simulink model "strapnav"  (Simulink 7.9)
settings: Solver=ode45  StartTime=0.0  StopTime=10.0  RelTol=1e-3
undefined symbols (not defined in the file or in its folder): dcm2lat, dcm2lon
libraries: simulink x2, strapnavlib x1
settings Model: Creator=mcar  LastModifiedBy=1104070  ExtModeAutoUpdateStatusClock=off  BufferReuse=off
settings DataIOCC: SaveFormat=StructureWithTime  SignalLoggingName=sigsOut
settings OptimizationCC: BooleanDataType=off  OptimizeBlockIOStorage=off  BufferReuse=off  ExpressionFolding=off  LocalBlockOutputs=off
settings DebuggingCC: SaveWithParameterizedLinksMsg=none  SignalResolutionControl=TryResolveAllWithWarning  SolverPrmCheckMsg=none  MultiTaskDSMMsg=warning  MultiTaskCondExecSysMsg=none  StrictBusMsg=None
settings HardwareCC: TargetUnknown=on
settings RTWCC: IncludeERTFirstTime=on
settings GRTTargetCC: CombineOutputUpdateFcns=off  GRTInterface=on

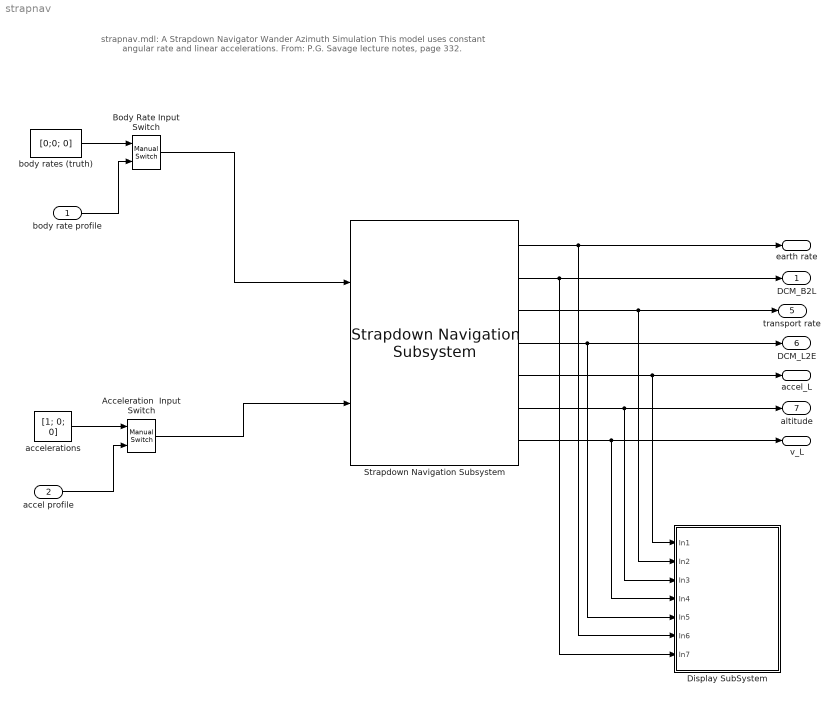
== system strapnav ==
  note: strapnav.mdl: A Strapdown Navigator Wander Azimuth Simulation
      | This model uses constant angular rate and linear accelerations.
      | From: P.G. Savage lecture notes, page 332.
  body rate profile : Inport
  accel profile : Inport  Port=2
  Acceleration  Input Switch : simulink/Signal Routing/Manual Switch  sw=1  action=0  varsize=off
  Body Rate Input Switch : simulink/Signal Routing/Manual Switch  sw=1  action=0  varsize=off
  Display SubSystem : Subsystem
  Strapdown Navigation Subsystem : strapnavlib/Strapdown Navigation Subsystem
  accelerations : Constant  Value=[1; 0; 0]  VectorParams1D=off
  body rates (truth) : Constant  Value=[0;0; 0]  VectorParams1D=off
  DCM_B2L : Outport
  accel_L : Outport  Port=2
  v_L : Outport  Port=3
  earth rate : Outport  Port=4
  transport rate : Outport  Port=5
  DCM_L2E : Outport  Port=6
  altitude : Outport  Port=7
  wires:
  body rates (truth)/1 -> Body Rate Input Switch/1
  Body Rate Input Switch/1 -> Strapdown Navigation Subsystem/1
  body rate profile/1 -> Body Rate Input Switch/2
  accelerations/1 -> Acceleration  Input Switch/1
  Acceleration  Input Switch/1 -> Strapdown Navigation Subsystem/2
  accel profile/1 -> Acceleration  Input Switch/2
  Strapdown Navigation Subsystem/1 -> earth rate/1, Display SubSystem/6(In6)
  Strapdown Navigation Subsystem/3 -> transport rate/1, Display SubSystem/2(In2)
  Strapdown Navigation Subsystem/4 -> DCM_L2E/1, Display SubSystem/5(In5)
  Strapdown Navigation Subsystem/5 -> accel_L/1, Display SubSystem/1(In1)
  Strapdown Navigation Subsystem/6 -> altitude/1, Display SubSystem/3(In3)
  Strapdown Navigation Subsystem/7 -> v_L/1, Display SubSystem/4(In4)
  Strapdown Navigation Subsystem/2 -> DCM_B2L/1, Display SubSystem/7(In7)

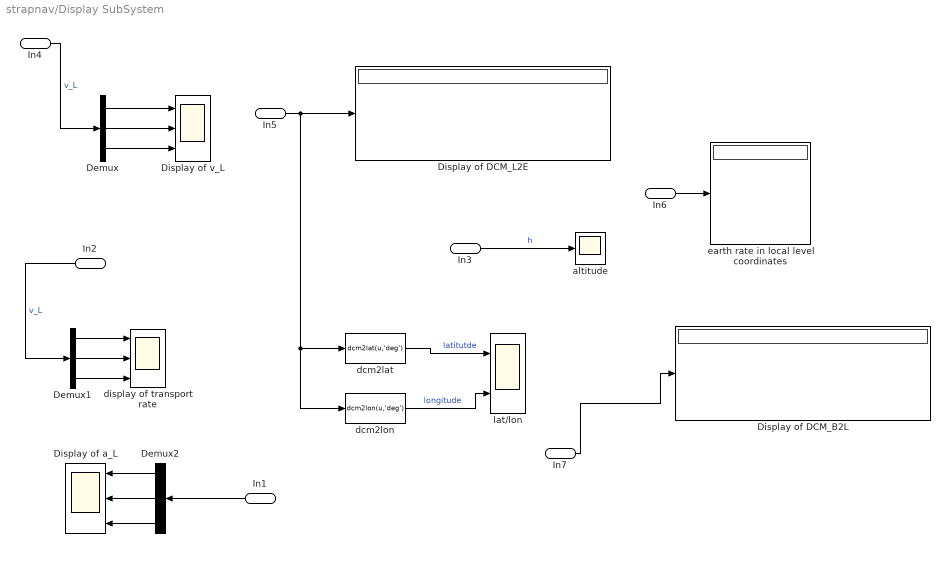
== system strapnav/Display SubSystem ==
  In1 : Inport
  In2 : Inport  Port=2
  In3 : Inport  Port=3
  In4 : Inport  Port=4
  In5 : Inport  Port=5
  In6 : Inport  Port=6
  In7 : Inport  Port=7
  Demux : Demux  Outputs=3
  Demux1 : Demux  Outputs=3
  Demux2 : Demux  Outputs=3
  Display of DCM_B2L : Display
  Display of DCM_L2E : Display
  Display of a_L : Scope  NumInputPorts=3
      settings: YMin=-5~-5~-5  YMax=5~5~5  SaveName=ScopeData2
  Display of v_L : Scope  NumInputPorts=3
      settings: YMin=-0.1~0~-2.5e-09  YMax=0.1~0.2~1.5e-08  SaveName=ScopeData4
  altitude : Scope
      settings: YMin=-1  YMax=1
  dcm2lat : MATLABFcn  MATLABFcn=dcm2lat(u,'deg')
  dcm2lon : MATLABFcn  MATLABFcn=dcm2lon(u,'deg')
  display of transport rate : Scope  NumInputPorts=3
      settings: YMin=-5~-5~-5  YMax=5~5~5  SaveName=ScopeData3
  earth rate in local level coordinates : Display
  lat/lon : Scope  NumInputPorts=2
      settings: YMin=-5~-5  YMax=5~5
  wires:
  In2/1 -> Demux1/1  "v_L"
  Demux1/1 -> display of transport rate/1
  Demux1/2 -> display of transport rate/2
  Demux1/3 -> display of transport rate/3
  In4/1 -> Demux/1  "v_L"
  Demux/1 -> Display of v_L/1
  Demux/2 -> Display of v_L/2
  Demux/3 -> Display of v_L/3
  dcm2lat/1 -> lat/lon/1  "latitutde"
  dcm2lon/1 -> lat/lon/2  "longitude"
  In5/1 -> Display of DCM_L2E/1, dcm2lat/1, dcm2lon/1
  In7/1 -> Display of DCM_B2L/1
  In6/1 -> earth rate in local level coordinates/1
  In3/1 -> altitude/1  "h"
  In1/1 -> Demux2/1
  Demux2/1 -> Display of a_L/1
  Demux2/2 -> Display of a_L/2
  Demux2/3 -> Display of a_L/3
